simulink model "Mini_Project"  (R2023a)
settings: Solver=FixedStepAuto  StartTime=0.0  StopTime=0.01  FixedStep=0.01  RelTol=1e-3
values from neighbouring files (symbols this model uses):
  Left_Turn_AngularLimit = -120.0    [MP_VDD.sldd]
  LeftTurn_RoadSign = -120.0    [MP_VDD.sldd]
  Right_Turn_AngularLimit = 30.0    [MP_VDD.sldd]
  RightTurn_RoadSign = 30.0    [MP_VDD.sldd]
  Straight_Drive_Steering_Angle = 0.0    [MP_VDD.sldd]
  Straight_RoadSign = 0.0    [MP_VDD.sldd]
libraries: simulink x3
settings Model: DataDictionary=MP_VDD.sldd  EnableAccessToBaseWorkspace=off  Creator=todka  LastModifiedBy=shilp
settings SolverCC: AlgebraicLoopSolver=TrustRegion
settings OptimizationCC: DefaultParameterBehavior=Inlined  EnhancedBackFolding=on  PassReuseOutputArgsAs=Individual arguments  ZeroExternalMemoryAtStartup=off  ZeroInternalMemoryAtStartup=off  OptimizeBlockOrder=speed  DifferentSizesBufferReuse=on  OptimizationCustomize=off  EfficientTunableParamExpr=on
settings DebuggingCC: SignalInfNanChecking=error  CheckMatrixSingularityMsg=error  IntegerOverflowMsg=error  ParameterTunabilityLossMsg=error  UnconnectedInputMsg=warning  UnconnectedOutputMsg=warning  UnconnectedLineMsg=warning  UniqueDataStoreMsg=warning  StrictBusMsg=ErrorOnBusTreatedAsVector  IntegerSaturationMsg=error
settings ModelReferenceCC: EnableRefExpFcnMdlSchedulingChecks=on
settings SFSimCC: MATLABDynamicMemAlloc=off
settings RTWCC: Description=Embedded Coder  SystemTargetFile=ert.tlc  TemplateMakefile=ert_default_tmf
settings CodeAppCC: ForceParamTrailComments=on  IgnoreCustomStorageClasses=off  OperatorAnnotations=on  SimulinkDataObjDesc=on  SFDataObjDesc=on  InsertBlockDesc=on
settings ERTTargetCC: TargetLangStandard=C99 (ISO)  GenerateSampleERTMain=on  InlinedParameterPlacement=NonHierarchical  ERTCustomFileTemplate=example_file_process.tlc

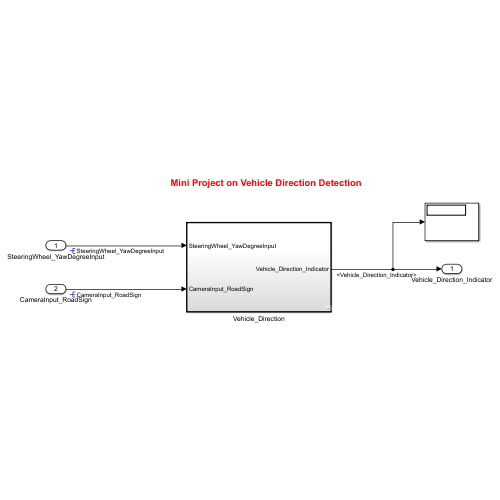
[thumbnail: Simulink's stored preview of the top-level diagram]
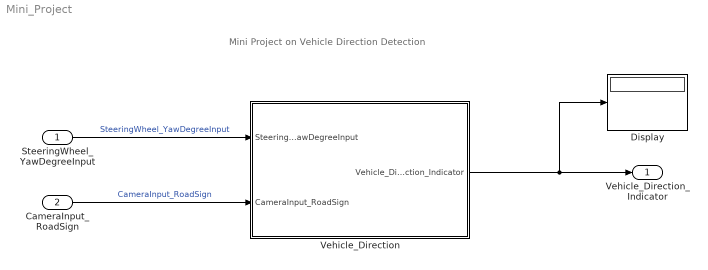
== system Mini_Project ==
  note: Mini Project on Vehicle Direction Detection
  SteeringWheel_YawDegreeInput : Inport
  CameraInput_RoadSign : Inport  Port=2
  Display : Display
  Vehicle_Direction : Subsystem  TreatAsAtomicUnit=on
  Vehicle_Direction_Indicator : Outport
  wires:
  SteeringWheel_YawDegreeInput/1 -> Vehicle_Direction/1(SteeringWheel_YawDegreeInput)  "SteeringWheel_YawDegreeInput"
  CameraInput_RoadSign/1 -> Vehicle_Direction/2(CameraInput_RoadSign)  "CameraInput_RoadSign"
  Vehicle_Direction/1(Vehicle_Direction_Indicator) -> Display/1, Vehicle_Direction_Indicator/1

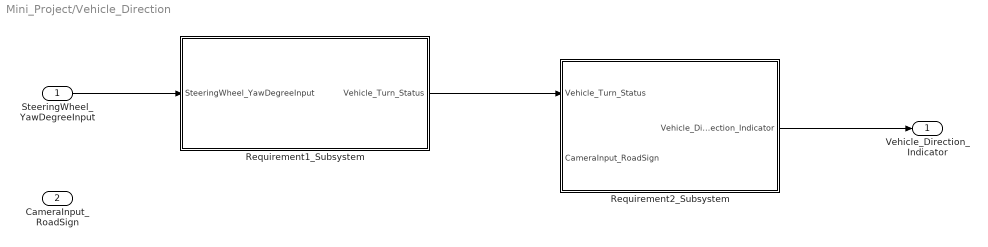
== system Mini_Project/Vehicle_Direction ==
  SteeringWheel_YawDegreeInput : Inport
  CameraInput_RoadSign : Inport  Port=2
  Requirement1_Subsystem : Subsystem
  Requirement2_Subsystem : Subsystem
  Vehicle_Direction_Indicator : Outport
  wires:
  SteeringWheel_YawDegreeInput/1 -> Requirement1_Subsystem/1(SteeringWheel_YawDegreeInput)
  Requirement2_Subsystem/1(Vehicle_Direction_Indicator) -> Vehicle_Direction_Indicator/1
  Requirement1_Subsystem/1(Vehicle_Turn_Status) -> Requirement2_Subsystem/1(Vehicle_Turn_Status)

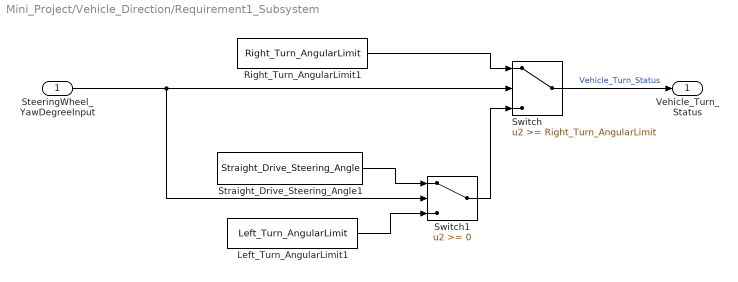
== system Mini_Project/Vehicle_Direction/Requirement1_Subsystem ==
  SteeringWheel_YawDegreeInput : Inport
  Left_Turn_AngularLimit1 : Constant  Value=Left_Turn_AngularLimit
  Right_Turn_AngularLimit1 : Constant  Value=Right_Turn_AngularLimit
  Straight_Drive_Steering_Angle1 : Constant  Value=Straight_Drive_Steering_Angle
  Switch : Switch  Threshold=Right_Turn_AngularLimit  SaturateOnIntegerOverflow=off  InputSameDT=off
  Switch1 : Switch  SaturateOnIntegerOverflow=off  InputSameDT=off
  Vehicle_Turn_Status : Outport
  wires:
  SteeringWheel_YawDegreeInput/1 -> Switch1/2, Switch/2
  Switch1/1 -> Switch/3
  Switch/1 -> Vehicle_Turn_Status/1  "Vehicle_Turn_Status"
  Right_Turn_AngularLimit1/1 -> Switch/1
  Left_Turn_AngularLimit1/1 -> Switch1/3
  Straight_Drive_Steering_Angle1/1 -> Switch1/1

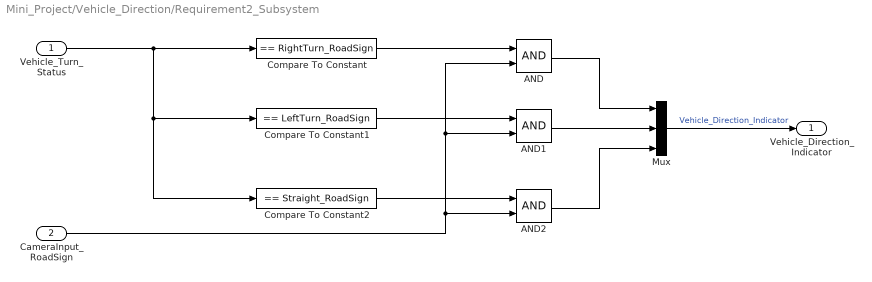
== system Mini_Project/Vehicle_Direction/Requirement2_Subsystem ==
  Vehicle_Turn_Status : Inport
  CameraInput_RoadSign : Inport  Port=2
  AND : Logic  OutDataTypeStr=boolean
  AND1 : Logic  OutDataTypeStr=boolean
  AND2 : Logic  OutDataTypeStr=boolean
  Compare To Constant : simulink/Logic and Bit Operations/Compare To Constant  relop===  const=RightTurn_RoadSign  OutDataTypeStr=boolean
  Compare To Constant1 : simulink/Logic and Bit Operations/Compare To Constant  relop===  const=LeftTurn_RoadSign  OutDataTypeStr=boolean
  Compare To Constant2 : simulink/Logic and Bit Operations/Compare To Constant  relop===  const=Straight_RoadSign  OutDataTypeStr=boolean
  Mux : Mux  Inputs=3
  Vehicle_Direction_Indicator : Outport
  wires:
  Vehicle_Turn_Status/1 -> Compare To Constant/1, Compare To Constant2/1, Compare To Constant1/1
  Compare To Constant/1 -> AND/1
  CameraInput_RoadSign/1 -> AND/2, AND1/2, AND2/2
  Compare To Constant1/1 -> AND1/1
  Compare To Constant2/1 -> AND2/1
  AND/1 -> Mux/1
  AND1/1 -> Mux/2
  AND2/1 -> Mux/3
  Mux/1 -> Vehicle_Direction_Indicator/1  "Vehicle_Direction_Indicator"
